simulink model "Stabilizer_QDrone"  (Simulink 9.3)
settings: Solver=ode2  StartTime=0.0  StopTime=inf  FixedStep=0.001  RelTol=1e-3  EnableMultiTasking=on
model workspace (MAT data in the model file):
  Sig = Simulink.Signal
  Sig.DataType = 'auto'
  Sig.Dimensions = -1
  Sig.DimensionsMode = 'auto'
  Sig.Complexity = 'auto'
  Sig.SampleTime = -1
  Sig.SamplingMode = 'auto'
  video_step_size = 0.06
undefined symbols (not defined in the file): datetime, HIL, m, qc_get_step_size, QDrone_, saved_data, Stabilizer_
libraries: quarc_library x28, simulink_extras x5, simulink x4
settings Model: Creator=Admin  LastModifiedBy=user  SimulationMode=external
settings SolverCC: PositivePriorityOrder=on
settings DataIOCC: SaveFormat=Dataset  SignalLoggingSaveFormat=Dataset
settings OptimizationCC: LifeSpan=auto
settings DebuggingCC: UnderspecifiedInitializationDetection=Simplified  MergeDetectMultiDrivingBlocksExec=error  ParameterPrecisionLossMsg=none  FcnCallInpInsideContextMsg=error
settings HardwareCC: ProdBitPerLong=64  ProdBitPerPointer=64  ProdBitPerSizeT=64  ProdBitPerPtrDiffT=64  ProdLargestAtomicFloat=Float  ProdIntDivRoundTo=Zero  ProdEndianess=LittleEndian  ProdWordSize=64  ProdHWDeviceType=Intel->x86-64 (Linux 64)
settings ModelReferenceCC: PropagateSignalLabelsOutOfModel=on
settings RTWCC: SystemTargetFile=quarc_linux_x64.tlc  TemplateMakefile=quarc_default_tmf  Description=QUARC Linux x64 Target (QDrone) Using Toolchain  Toolchain=QUARC linux_x64 | gmake (64-bit Windows)  BuildConfiguration=Faster Runs
settings STFCustomTargetCC: TargetPreCompLibLocation=C:\PROGRA~3\QUARC\lib\2019a\LINUX_~1\release  ConcurrentExecutionCompliant=on  SystemTargetFile=quarc_linux_x64.tlc
settings GRTTargetCC: TargetPreCompLibLocation=C:\PROGRA~3\QUARC\lib\2019a\LINUX_~1\release  ParMdlRefBuildCompliant=off  CompOptLevelCompliant=off  MatFileLogging=off  CPPClassGenCompliant=off  UseToolchainInfoCompliant=off  ExtMode=on  ExtModeMexFile=quarc_comm  ExtModeMexArgs='-w -d /tmp -uri %u -URI_Host tcpip://192.168.2.5:18001', 'tcpip://192.168.2.30:17001?retries=10', 'tcpip://192.168.2.30:17000'
settings ConfigComp: CovHtmlReporting=off

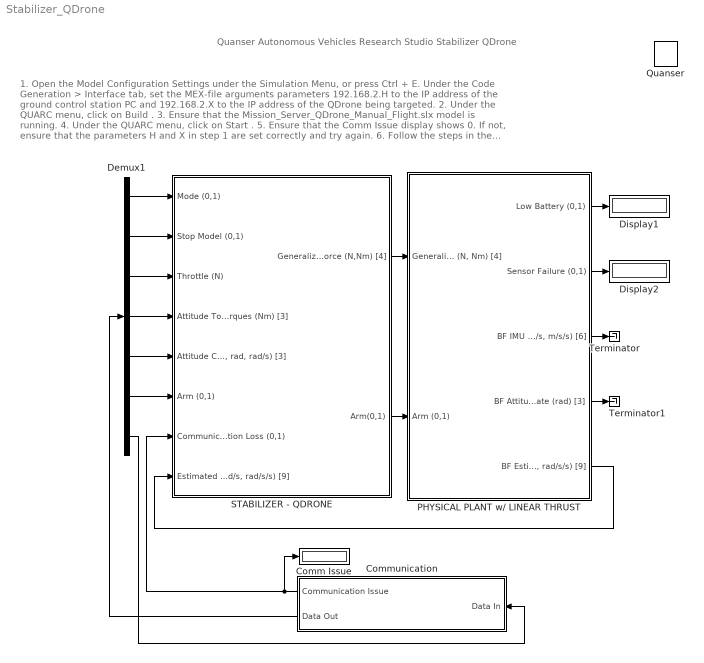
== system Stabilizer_QDrone ==
  note: Quanser Autonomous Vehicles Research Studio
      | Stabilizer QDrone
  note: 1. Open the Model Configuration Settings under the Simulation Menu, or press Ctrl + E. Under the Code Generation > Interface tab, set the MEX-file arguments parameters 192.168.2.H to the IP address of the ground control station PC and 192.168.2.X to the IP address of the QDrone being targeted.
      | 2. Under the QUARC menu, click on Build .
      | 3. Ensure that the Mission_Server_QDrone_Manual_Flight.slx model is running.
      | 4. Under the QUARC menu, click on Start .
      | 5. Ensure that the Comm Issue display shows 0. If not, ensure that the parameters H and X in step 1 are set correctly and try again.
      | 6. Follow the steps in the model to fly the drone.
      | 7. When flying is complete, stop this model first, and then the stop the Mission_Server_QDrone_Manual_Flight.slx model.
  Comm Issue : Display
  Communication : Subsystem
  Demux1 : Demux  Outputs=[1 1 1 3 3 1 1]
  Display1 : Display
      settings: Decimation=100
  Display2 : Display
      settings: Decimation=100
  PHYSICAL PLANT w/ LINEAR THRUST : Subsystem
  Quanser : quarc_library/Logos/Quanser
  STABILIZER - QDRONE : Subsystem
  Terminator : Terminator
  Terminator1 : Terminator
  wires:
  Demux1/7 -> Communication/1(Data In)
  Communication/2(Data Out) -> Demux1/1
  STABILIZER - QDRONE/1(Generalized  Force (N,Nm) [4]) -> PHYSICAL PLANT w/ LINEAR THRUST/1("Generalized Force (N, Nm) [4]")
  STABILIZER - QDRONE/2(Arm(0,1)) -> PHYSICAL PLANT w/ LINEAR THRUST/2(Arm (0,1))
  Communication/1(Communication Issue) -> Comm Issue/1, STABILIZER - QDRONE/7(Communication Loss (0,1))
  Demux1/1 -> STABILIZER - QDRONE/1(Mode (0,1))
  Demux1/2 -> STABILIZER - QDRONE/2(Stop Model (0,1))
  Demux1/3 -> STABILIZER - QDRONE/3(Throttle (N))
  Demux1/4 -> STABILIZER - QDRONE/4(Attitude Torques (Nm) [3])
  Demux1/5 -> STABILIZER - QDRONE/5("Attitude Commands (rad, rad, rad/s) [3]")
  PHYSICAL PLANT w/ LINEAR THRUST/5("BF Estimated Attitude (rad, rad/s, rad/s/s) [9]") -> STABILIZER - QDRONE/8("Estimated Attitude (rad, rad/s, rad/s/s) [9]")
  Demux1/6 -> STABILIZER - QDRONE/6(Arm (0,1))
  PHYSICAL PLANT w/ LINEAR THRUST/1(Low Battery (0,1)) -> Display1/1
  PHYSICAL PLANT w/ LINEAR THRUST/2(Sensor Failure (0,1)) -> Display2/1
  PHYSICAL PLANT w/ LINEAR THRUST/3("BF IMU Data (rad/s, m/s/s) [6]") -> Terminator/1
  PHYSICAL PLANT w/ LINEAR THRUST/4(" BF Attitude Estimate (rad) [3]") -> Terminator1/1

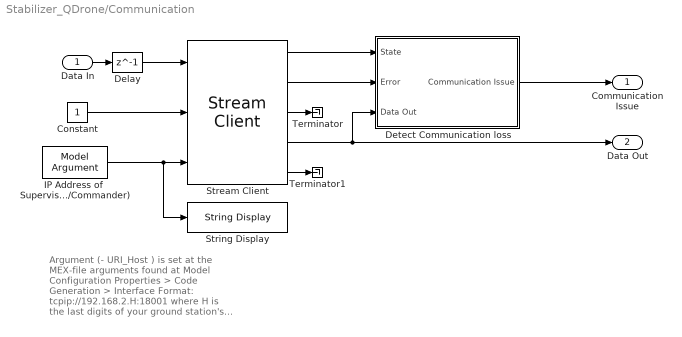
== system Stabilizer_QDrone/Communication ==
  note: Argument (- URI_Host ) is set at the MEX-file arguments found at Model Configuration Properties > Code Generation > Interface
      |
      | Format:
      | tcpip://192.168.2.H:18001
      | where H is the last digits of your ground station's IP address (use ipconfig in a command prompt to find it out).
  Data In : Inport
  Constant : Constant
  Delay : Delay  DelayLength=1
  Detect Communication loss : Subsystem
  IP Address of  Supervisory Model (Mission Operator/Commander) : quarc_library/Sources/Signals/Model Argument  argument_name=URI_Host  has_value=on  data_type_mode=Specify via dialog  data_type=char  max_length=80  variable_size=off
      settings: AttributesFormatString=(-%<argument_name>)  SourceProductName=QUARC Targets
  Stream Client : quarc_library/Communications/Basic/Stream Client  uri_source=External input port  uri=tcpip://localhost:18999  apply_uri_to_all_configs=on  send_buffer_size=1460  receive_buffer_size=1460  byte_order=little endian (Intel - LSB first)  optimization=Minimum latency  send_options=Send most recent data  receive_options=Receive most recent data  default_value=zeros(1,11)  sample_time=qc_get_step_size  active=off  implementation=Use blocking I/O in a separate thread  send_fifo_size=1  receive_fifo_size=1  send_priority=0  receive_priority=0  send_dimensions=off  receive_dimensions=off  max_dimensions=-1  data_type=Inherited via back propagation  type_expr=BusObject
      settings: SourceProductName=The database C:\Users\user\AppData\Roaming\MathWorks\MATLAB\R2017a\slblocks_master.db is locked, or a table in the database is locked. (database is locked)
  String Display : quarc_library/Strings/String Display  alignment=center  display_mode=Single line  sample_time=-1  use_new=off
      settings: SourceProductName=QUARC Targets
  Terminator : Terminator
  Terminator1 : Terminator
  Communication Issue : Outport
  Data Out : Outport  Port=2
  wires:
  Stream Client/5 -> Terminator1/1
  Constant/1 -> Stream Client/2
  Stream Client/3 -> Terminator/1
  IP Address of  Supervisory Model (Mission Operator/Commander)/1 -> String Display/1, Stream Client/3
  Stream Client/1 -> Detect Communication loss/1(State)
  Stream Client/2 -> Detect Communication loss/2(Error)
  Stream Client/4 -> Detect Communication loss/3(Data Out), Data Out/1
  Data In/1 -> Delay/1
  Delay/1 -> Stream Client/1
  Detect Communication loss/1(Communication Issue) -> Communication Issue/1

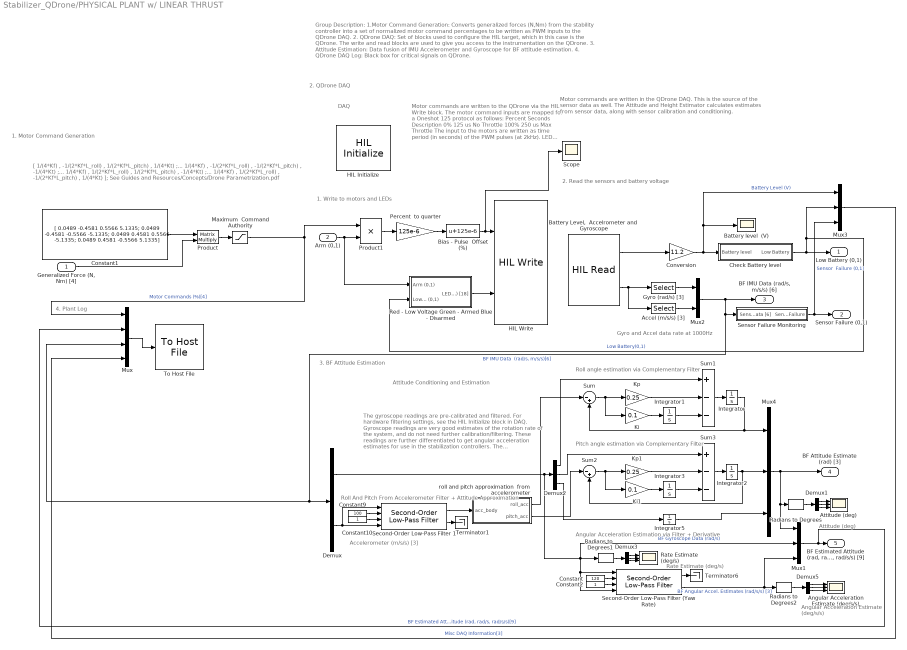
== system Stabilizer_QDrone/PHYSICAL PLANT w/ LINEAR THRUST ==
  note: Rate Estimate (deg/s)
  note: Accelerometer (m/s/s) [3]
  note: Roll And Pitch From Accelerometer Filter + Attitude Approximation
  note: Attitude Conditioning and Estimation
  note: Pitch angle estimation via Complementary Filter
  note: Roll angle estimation via Complementary Filter
  note: The gyroscope readings are pre-calibrated and filtered. For hardware filtering settings, see the HIL Initialize block in DAQ. Gyroscope readings are very good estimates of the rotation rate of the system, and do not need further calibration/filtering. These readings are further differentiated to get angular acceleration estimates for use in the stabilization controllers.
      |
      | The accelerometer readings in body reference frame are used to calculate a roll and pitch approximation. This is based on the knowledge that the gravity vector points straight down.
  note: Angular Acceleration Estimation via Filter + Derivative
  note: DAQ
  note: Motor commands are written to the QDrone via the HIL Write block. The motor command inputs are mapped for a Oneshot 125 protocol as follows:
      |
      | Percent Seconds Description
      | 0% 125 us No Throttle
      | 100% 250 us Max Throttle
      |
      | The input to the motors are written as time period (in seconds) of the PWM pulses (at 2kHz).
      |
      | LED colors can be set using a simple 3x1 ON (1) and OFF (0) vector (RGB mode).
  note: 1. Write to motors and LEDs
  note: 2. Read the sensors and battery voltage
  note: Gyro and Accel data rate at 1000Hz
  note: 1. Motor Command Generation
  note: Motor commands are written in the QDrone DAQ. This is the source of the sensor data as well. The Attitude and Height Estimator calculates estimates from sensor data, along with sensor calibration and conditioning.
  note: Angular Acceleration
      | Estimate (deg/s/s)
  note: Attitude (deg)
  note: [ 1/(4*Kf) , -1/(2*Kf*L_roll) , 1/(2*Kf*L_pitch) , 1/(4*Kt) ;...
      | 1/(4*Kf) , -1/(2*Kf*L_roll) , -1/(2*Kf*L_pitch) , -1/(4*Kt) ;...
      | 1/(4*Kf) , 1/(2*Kf*L_roll) , 1/(2*Kf*L_pitch) , -1/(4*Kt) ;...
      | 1/(4*Kf) , 1/(2*Kf*L_roll) , -1/(2*Kf*L_pitch) , 1/(4*Kt) ];
      |
      | See Guides and Resources/Concepts/Drone Parametrization.pdf
  note: 4. Plant Log
  note: Group Description:
      |
      | 1.Motor Command Generation: Converts generalized forces (N,Nm) from the stability controller into a set of normalized motor command percentages to be written as PWM inputs to the QDrone DAQ.
      | 2. QDrone DAQ: Set of blocks used to configure the HIL target, which in this case is the QDrone. The write and read blocks are used to give you access to the instrumentation on the QDrone.
      | 3. Attitude Estimation: Data fusion of IMU Accelerometer and Gyroscope for BF attitude estimation.
      | 4. QDrone DAQ Log: Black box for critical signals on QDrone.
  note: 2. QDrone DAQ
  note: 3. BF Attitude Estimation
  "Generalized Force (N, Nm) [4]" : Inport
  Arm (0,1) : Inport  Port=2
  Accel (m/s/s) [3] : Selector  InputPortWidth=6  IndexOptions=Index vector (dialog)  Indices=[4:6]  OutputSizes=1
  Angular Acceleration Estimate (deg/s/s) : Scope  NumInputPorts=3
  Attitude (deg) : Scope  NumInputPorts=3
  "Battery Level,  Accelrometer and  Gyroscope" : quarc_library/Data Acquisition/Generic/Immediate I//O/HIL Read  Priority=1  object_name=HIL-1  analog_channels=[4]  encoder_channels=[]  digital_channels=[]  other_channels=[3000:3002 4000:4002]  sample_time=qc_get_step_size  active=on  vector_output=on  data_type_mode=Inherit via back propagation  encoder_data_type=double  digital_data_type=boolean
      settings: SourceProductName=The database C:\Users\user\AppData\Roaming\MathWorks\MATLAB\R2017a\slblocks_master.db is locked, or a table in the database is locked. (database is locked)
  Battery level  (V) : Scope
  Bias - Pulse  Offset (%) : Bias  Bias=125e-6
  Check Battery level : Subsystem
  Constant : Constant  Value=120
  Constant1 : Constant  Value=|
      | [ 0.0489   -0.4581    0.5566    5.1335;
      |   0.0489   -0.4581   -0.5566   -5.1335;
      |   0.0489    0.4581    0.5566   -5.1335;
      |   0.0489    0.4581   -0.5566    5.1335]
  Constant10 : Constant
  Constant2 : Constant
  Constant9 : Constant  Value=100
  Conversion : Gain  Gain=11.2
  Demux : Demux  Outputs=[3 3]
  Demux{1..3,5} (4 alike) : Demux  Outputs=3
  Gyro (rad/s) [3] : Selector  InputPortWidth=6  IndexOptions=Index vector (dialog)  Indices=[1:3]  OutputSizes=1
  HIL Initialize : quarc_library/Data Acquisition/Generic/Configuration/HIL Initialize  object_name=HIL-1  board_type=qdrone  board_number=0  board_options=gyro_fs=2000;gyro_rate=1000;gyro_os=4;accel_fs=16;accel_rate=400;accel_os=4;baro_os=4096  exclusive=off  active=on  hardware_clocks=[]  clock_modes=[]  initial_clock_frequencies=[]  set_clock_params_at_start=off  set_clock_params_at_switch_in=off  set_clock_frequencies_at_start=off  set_clock_frequencies_at_switch_in=off  analog_input_channels=[0:4]  analog_input_configurations=[]  analog_input_maximums=[3.3]  analog_input_minimums=[0]  set_analog_input_params_at_start=off  set_analog_input_params_at_switch_in=off  analog_output_channels=[]  analog_output_maximums=[]  analog_output_minimums=[]  initial_analog_outputs=[]  final_analog_outputs=[]  watchdog_analog_outputs=[]  set_analog_output_params_at_start=off  set_analog_output_params_at_switch_in=off  set_analog_outputs_at_start=off  set_analog_outputs_at_switch_in=off  set_analog_outputs_at_terminate=off  set_analog_outputs_at_switch_out=off  set_analog_outputs_on_watchdog=off  digital_input_channels=[]  digital_output_channels=[5:7 9:23]  digital_output_configuration=[]  initial_digital_outputs=[0]  final_digital_outputs=[0]  watchdog_digital_outputs=[]  set_digital_output_params_at_start=off  set_digital_output_params_at_switch_in=off  set_digital_outputs_at_start=on  set_digital_outputs_at_switch_in=off  set_digital_outputs_at_terminate=on  set_digital_outputs_at_switch_out=off  set_digital_outputs_on_watchdog=off  encoder_channels=[0:2]  quadrature=[4]  encoder_filter_frequency=50e6/1  initial_encoder_counts=[0]  set_encoder_params_at_start=on  set_encoder_params_at_switch_in=off  set_encoder_counts_at_start=on  set_encoder_counts_at_switch_in=off  pwm_channels=[0:3]  pwm_modes=[4]  pwm_frequency=2000  pwm_configuration=[0]  pwm_alignment=[0]  pwm_polarity=[1]  pwm_leading_deadband=[]  pwm_trailing_deadband=[]  initial_pwm_outputs=[0]  final_pwm_outputs=[0]  watchdog_pwm_outputs=[0]  set_pwm_params_at_start=on  set_pwm_params_at_switch_in=off  set_pwm_outputs_at_start=on  set_pwm_outputs_at_switch_in=off  set_pwm_outputs_at_terminate=on  set_pwm_outputs_at_switch_out=off  set_pwm_outputs_on_watchdog=off  other_output_channels=[]  initial_other_outputs=[]  final_other_outputs=[]  watchdog_other_outputs=[]  set_other_outputs_at_start=off  set_other_outputs_at_switch_in=off  set_other_outputs_at_terminate=off  set_other_outputs_at_switch_out=off  set_other_outputs_on_watchdog=off
      settings: SourceProductName=The database C:\Users\user\AppData\Roaming\MathWorks\MATLAB\R2017a\slblocks_master.db is locked, or a table in the database is locked. (database is locked)
  HIL Write : quarc_library/Data Acquisition/Generic/Immediate I//O/HIL Write  object_name=HIL-1  analog_channels=[]  pwm_channels=[0:3]  digital_channels=[5:7 9:23]  other_channels=[]  sample_time=-1  active=off  vector_input=on
      settings: SourceProductName=The database C:\Users\user\AppData\Roaming\MathWorks\MATLAB\R2017a\slblocks_master.db is locked, or a table in the database is locked. (database is locked)
  Integrator{,1..3,5} (5 alike) : Integrator
  Ki : Gain  Gain=0.1
  Ki1 : Gain  Gain=0.1
  Kp : Gain  Gain=0.25
  Kp1 : Gain  Gain=0.25
  "Maximum  Command Authority " : Saturate  UpperLimit=[1 1 1 1]  LowerLimit=[0 0 0 0]
  Mux : Mux
  Mux1 : Mux  Inputs=3
  Mux2 : Mux  Inputs=2
  Mux3 : Mux  Inputs=3
  Mux4 : Mux  Inputs=3
  Percent  to quarter : Gain  Gain=125e-6
  Product : Product  Multiplication=Matrix(*)
  Product1 : Product
  Radians to Degrees : simulink_extras/Transformations/Radians to Degrees
  Radians to Degrees1 : simulink_extras/Transformations/Radians to Degrees
  Radians to Degrees2 : simulink_extras/Transformations/Radians to Degrees
  Rate Estimate (deg/s) : Scope  NumInputPorts=3
  Red - Low Voltage Green - Armed Blue - Disarmed : Subsystem
  Scope : Scope
  Second-Order Low-Pass Filter (Yaw Rate) : quarc_library/Continuous/Second-Order Low-Pass Filter  params_source=External (input ports)  input_width=200  input_zeta=1  input_init=0
      settings: SourceProductName=The database C:\Users\user\AppData\Roaming\MathWorks\MATLAB\R2017a\slblocks_master.db is locked, or a table in the database is locked. (database is locked)
  Second-Order Low-Pass Filter 1 : quarc_library/Continuous/Second-Order Low-Pass Filter  params_source=External (input ports)  input_width=50  input_zeta=1  input_init=0
      settings: SourceProductName=The database C:\Users\user\AppData\Roaming\MathWorks\MATLAB\R2017a\slblocks_master.db is locked, or a table in the database is locked. (database is locked)
  Sensor Failure Monitoring : Subsystem
  Sum : Sum  Inputs=|-+
  Sum1 : Sum  Inputs=+--
  Sum2 : Sum  Inputs=|-+
  Sum3 : Sum  Inputs=+--
  Terminator1 : Terminator
  Terminator6 : Terminator
  To Host File : quarc_library/Sinks/To Host/To Host File  file_name=saved_data/%m/QDrone_%{char(datetime)}.mat  variable_name=QDrone_data  decimation=1  sample_time=-1  file_format=MAT-file v.5  options=No header or footer  append=off  final_file_name=saved_data/Stabilizer_QDrone/QDrone_05-Nov-2026 13-08-41.mat  bitrate=2000000
      settings: SourceProductName=The database C:\Users\user\AppData\Roaming\MathWorks\MATLAB\R2017a\slblocks_master.db is locked, or a table in the database is locked. (database is locked)
  roll and pitch approximation  from accelerometer : MATLAB Function  TreatAsAtomicUnit=on
  Low Battery (0,1) : Outport
  Sensor Failure (0,1) : Outport  Port=2
  "BF IMU Data (rad/s, m/s/s) [6]" : Outport  Port=3
  " BF Attitude Estimate (rad) [3]" : Outport  Port=4
  "BF Estimated Attitude (rad, rad/s, rad/s/s) [9]" : Outport  Port=5
  wires:
  Mux3/1 -> Mux/4  "Misc DAQ Information[3]"
  Check Battery level/1(Low Battery) -> Low Battery (0,1)/1, Red - Low Voltage Green - Armed Blue - Disarmed/2(Low Battery (0,1)), Mux3/2  "Low Battery(0,1)"
  Arm (0,1)/1 -> Product1/2, Red - Low Voltage Green - Armed Blue - Disarmed/1(Arm (0,1))
  Mux1/1 -> "BF Estimated Attitude (rad, rad/s, rad/s/s) [9]"/1, Mux/2  "BF Estimated Attitude (rad, rad/s, rad/s/s)[9]"
  Demux3/1 -> Rate Estimate (deg/s)/1
  Demux3/2 -> Rate Estimate (deg/s)/2
  Radians to Degrees1/1 -> Demux3/1
  Demux/1 -> Demux2/1, Second-Order Low-Pass Filter (Yaw Rate)/1, Second-Order Low-Pass Filter (Yaw Rate)/4, Radians to Degrees1/1, Mux1/2  "BF Gyroscope Data (rad/s)"
  Demux3/3 -> Rate Estimate (deg/s)/3
  Second-Order Low-Pass Filter (Yaw Rate)/2 -> Mux1/3, Radians to Degrees2/1  "BF Angular Accel. Estimates (rad/s/s) [3]"
  Second-Order Low-Pass Filter 1/2 -> Terminator1/1
  roll and pitch approximation  from accelerometer/2(pitch_acc) -> Sum2/1
  Kp/1 -> Sum1/2
  Constant10/1 -> Second-Order Low-Pass Filter 1/3
  Demux/2 -> Second-Order Low-Pass Filter 1/4, Second-Order Low-Pass Filter 1/1
  Constant2/1 -> Second-Order Low-Pass Filter (Yaw Rate)/3
  Sum/1 -> Kp/1, Ki/1
  Demux2/3 -> Integrator5/1
  roll and pitch approximation  from accelerometer/1(roll_acc) -> Sum/1
  Second-Order Low-Pass Filter 1/1 -> roll and pitch approximation  from accelerometer/1(acc_body)
  Second-Order Low-Pass Filter (Yaw Rate)/1 -> Terminator6/1
  Constant9/1 -> Second-Order Low-Pass Filter 1/2
  Mux4/1 -> " BF Attitude Estimate (rad) [3]"/1, Mux1/1, Radians to Degrees/1
  Ki1/1 -> Integrator3/1
  Integrator1/1 -> Sum1/3
  Sum1/1 -> Integrator/1
  Sum3/1 -> Integrator2/1
  Sum2/1 -> Ki1/1, Kp1/1
  Kp1/1 -> Sum3/2
  Integrator/1 -> Mux4/1, Sum/2
  Constant/1 -> Second-Order Low-Pass Filter (Yaw Rate)/2
  Demux2/1 -> Sum1/1
  Ki/1 -> Integrator1/1
  Integrator5/1 -> Mux4/3
  Integrator2/1 -> Mux4/2, Sum2/2
  Integrator3/1 -> Sum3/3
  Demux2/2 -> Sum3/1
  Mux2/1 -> "BF IMU Data (rad/s, m/s/s) [6]"/1, Sensor Failure Monitoring/1(Sensor Data [6]), Demux/1, Mux/3  "BF IMU Data  (rad/s, m/s/s)[6]"
  Sensor Failure Monitoring/1(Sensor Failure) -> Mux3/3, Sensor Failure (0,1)/1  "Sensor  Failure (0,1)"
  Gyro (rad/s) [3]/1 -> Mux2/1
  "Battery Level,  Accelrometer and  Gyroscope"/1 -> Conversion/1
  "Battery Level,  Accelrometer and  Gyroscope"/2 -> Gyro (rad/s) [3]/1, Accel (m/s/s) [3]/1
  Percent  to quarter/1 -> Bias - Pulse  Offset (%)/1
  Bias - Pulse  Offset (%)/1 -> Scope/1, HIL Write/1
  Red - Low Voltage Green - Armed Blue - Disarmed/1(LEDs (%) [18]) -> HIL Write/2
  Product1/1 -> Percent  to quarter/1
  Accel (m/s/s) [3]/1 -> Mux2/2
  Mux/1 -> To Host File/1
  Product/1 -> "Maximum  Command Authority "/1
  "Generalized Force (N, Nm) [4]"/1 -> Product/2
  Constant1/1 -> Product/1
  Conversion/1 -> Battery level  (V)/1, Mux3/1, Check Battery level/1(Battery level)  "Battery Level (V)"
  "Maximum  Command Authority "/1 -> Product1/1, Mux/1  "Motor Commands (%)[4]"
  Radians to Degrees2/1 -> Demux5/1
  Radians to Degrees/1 -> Demux1/1
  Demux5/3 -> Angular Acceleration Estimate (deg/s/s)/3
  Demux5/2 -> Angular Acceleration Estimate (deg/s/s)/2
  Demux5/1 -> Angular Acceleration Estimate (deg/s/s)/1
  Demux1/3 -> Attitude (deg)/3
  Demux1/2 -> Attitude (deg)/2
  Demux1/1 -> Attitude (deg)/1

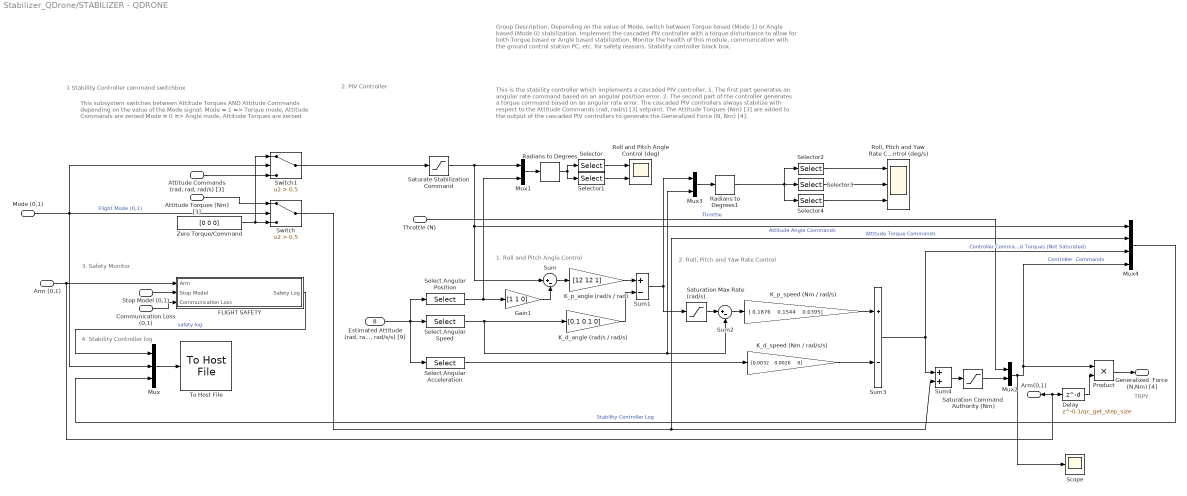
== system Stabilizer_QDrone/STABILIZER - QDRONE ==
  note: 2. PIV Controller
  note: 4. Stability Controller log
  note: 1 Stability Controller command switchbox
  note: Group Description:
      |
      | Depending on the value of Mode, switch between Torque based (Mode 1) or Angle based (Mode 0) stabilization.
      | Implement the cascaded PIV controller with a torque disturbance to allow for both Torque based or Angle based stabilization.
      | Monitor the health of this module, communication with the ground control station PC, etc. for safety reasons.
      | Stability controller black box.
  note: TRPY
  note: 2. Roll, Pitch and Yaw Rate Control
  note: 1. Roll and Pitch Angle Control
  note: This is the stability controller which implements a cascaded PIV controller.
      | 1. The first part generates an angular rate command based on an angular position error.
      | 2. The second part of the controller generates a torque command based on an angular rate error.
      |
      | The cascaded PIV controllers always stabilize with respect to the Attitude Commands (rad, rad/s) [3] setpoint. The Attitude Torques (Nm) [3] are added to the output of the cascaded PIV controllers to generate the Generalized Force (N, Nm) [4].
  note: This subsystem switches between Attitude Torques AND Attitude Commands depending on
      | the value of the Mode signal:
      | Mode = 1	=> 		Torque mode, Attitude Commands are zeroed
      | Mode = 0	=> 		Angle mode, Attitude Torques are zeroed
  note: 3. Safety Monitor
  Mode (0,1) : Inport
  Stop Model (0,1) : Inport  Port=2
  Throttle (N) : Inport  Port=3
  Attitude Torques (Nm) [3] : Inport  Port=4
  "Attitude Commands (rad, rad, rad/s) [3]" : Inport  Port=5
  Arm (0,1) : Inport  Port=6
  Communication Loss (0,1) : Inport  Port=7
  "Estimated Attitude (rad, rad/s, rad/s/s) [9]" : Inport  Port=8
  Delay : Delay  DelayLength=0.1/qc_get_step_size
  FLIGHT SAFETY : Subsystem
  Gain1 : Gain  Gain=[1 1 0]
  K_d_angle (rad/s / rad/s) : Gain  Gain=[0.1 0.1 0]
  K_d_speed (Nm / rad/s/s) : Gain  Gain="[0.0032    0.0026     0]"
  K_p_angle (rad/s / rad) : Gain  Gain=[12 12 1]
  K_p_speed (Nm / rad/s) : Gain  Gain="[ 0.1876    0.1544    0.0395]"
  Mux : Mux  Inputs=3
  Mux1 : Mux  Inputs=2
  Mux2 : Mux  Inputs=2
  Mux3 : Mux  Inputs=2
  Mux4 : Mux
  Product : Product
  Radians to Degrees : simulink_extras/Transformations/Radians to Degrees
  Radians to Degrees1 : simulink_extras/Transformations/Radians to Degrees
  Roll and Pitch Angle Control (deg) : Scope  NumInputPorts=2
  "Roll, Pitch and Yaw Rate Control (deg/s)" : Scope  NumInputPorts=3
  Saturate Stabilization Command : Saturate  UpperLimit=[pi/4 pi/4 10*pi/18]  LowerLimit=[-pi/4 -pi/4 -10*pi/18]
  Saturation Command  Authority (Nm) : Saturate  UpperLimit=[1.0915 0.8984 0.0984]  LowerLimit=-[1.0915 0.8984 0.0984]
  Saturation Max Rate  (rad/s) : Saturate  UpperLimit=10*pi/3*[1 1 1]  LowerLimit=-10*pi/3*[1 1 1]
  Scope : Scope
  Select Angular Acceleration : Selector  InputPortWidth=9  IndexOptions=Index vector (dialog)  Indices=[7:9]  OutputSizes=1
  Select Angular Speed : Selector  InputPortWidth=9  IndexOptions=Index vector (dialog)  Indices=[4:6]  OutputSizes=1
  Select Angular Position : Selector  InputPortWidth=9  IndexOptions=Index vector (dialog)  Indices=[1:3]  OutputSizes=1
  Selector : Selector  InputPortWidth=6  IndexOptions=Index vector (dialog)  Indices=[1 4]  OutputSizes=1
  Selector1 : Selector  InputPortWidth=6  IndexOptions=Index vector (dialog)  Indices=[2 5]  OutputSizes=1
  Selector2 : Selector  InputPortWidth=6  IndexOptions=Index vector (dialog)  Indices=[1 4]  OutputSizes=1
  Selector3 : Selector  InputPortWidth=6  IndexOptions=Index vector (dialog)  Indices=[2 5]  OutputSizes=1
  Selector4 : Selector  InputPortWidth=6  IndexOptions=Index vector (dialog)  Indices=[3 6]  OutputSizes=1
  Sum : Sum  Inputs=|+-
  Sum1 : Sum  Inputs=+-
  Sum2 : Sum  Inputs=|+-
  Sum3 : Sum  Inputs=+-
  Sum4 : Sum
  Switch : Switch  Criteria=u2 > Threshold  Threshold=0.5
  Switch1 : Switch  Criteria=u2 > Threshold  Threshold=0.5
  To Host File : quarc_library/Sinks/To Host/To Host File  file_name=saved_data/%m/Stabilizer_%{char(datetime)}.mat  variable_name=stabilizer_data  decimation=1  sample_time=-1  file_format=MAT-file v.5  options=No header or footer  append=off  final_file_name=saved_data/Stabilizer_QDrone/Stabilizer_05-Nov-2026 13-08-41.mat  bitrate=2000000
      settings: SourceProductName=The database C:\Users\user\AppData\Roaming\MathWorks\MATLAB\R2017a\slblocks_master.db is locked, or a table in the database is locked. (database is locked)
  Zero Torque/Command : Constant  Value=[0 0 0]
  Generalized  Force (N,Nm) [4] : Outport
  Arm(0,1) : Outport  Port=2
  wires:
  Product/1 -> Generalized  Force (N,Nm) [4]/1
  Stop Model (0,1)/1 -> FLIGHT SAFETY/2(Stop Model)
  Communication Loss (0,1)/1 -> FLIGHT SAFETY/3(Communication Loss)
  Mux/1 -> To Host File/1
  Mux4/1 -> Mux/3  "Stability Controller Log"
  Mode (0,1)/1 -> Switch/2, Switch1/2, Mux/2  "Flight Mode (0,1)"
  FLIGHT SAFETY/1(Safety Log) -> Mux/1  "safety log"
  K_p_speed (Nm / rad/s)/1 -> Sum3/1
  Sum/1 -> K_p_angle (rad/s / rad)/1
  K_d_speed (Nm / rad/s/s)/1 -> Sum3/2
  Arm (0,1)/1 -> Arm(0,1)/1, Delay/1, FLIGHT SAFETY/1(Arm)
  Mux3/1 -> Radians to Degrees1/1
  Sum1/1 -> Saturation Max Rate  (rad/s)/1, Mux3/1
  Saturate Stabilization Command/1 -> Mux1/1, Sum/1, Mux4/1  "Attitude Angle Commands"
  Mux2/1 -> Scope/1, Mux4/4, Product/1  "Controller  Commands"
  Select Angular Position/1 -> Mux1/2, Gain1/1
  Sum2/1 -> K_p_speed (Nm / rad/s)/1
  Throttle (N)/1 -> Mux2/1  "Throttle"
  Selector1/1 -> Roll and Pitch Angle Control (deg)/2
  Switch/1 -> Mux4/2, Sum4/2  "Attitude Torque Commands"
  Radians to Degrees1/1 -> Selector2/1, Selector4/1, Selector3/1
  "Estimated Attitude (rad, rad/s, rad/s/s) [9]"/1 -> Select Angular Position/1, Select Angular Acceleration/1, Select Angular Speed/1
  Mux1/1 -> Radians to Degrees/1
  Selector3/1 -> "Roll, Pitch and Yaw Rate Control (deg/s)"/2
  Sum4/1 -> Saturation Command  Authority (Nm)/1
  Sum3/1 -> Mux4/3, Sum4/1  "Controller Command Torques (Not Saturated)"
  Saturation Command  Authority (Nm)/1 -> Mux2/2
  Gain1/1 -> Sum/2
  Select Angular Acceleration/1 -> K_d_speed (Nm / rad/s/s)/1
  Switch1/1 -> Saturate Stabilization Command/1
  Saturation Max Rate  (rad/s)/1 -> Sum2/1
  Selector4/1 -> "Roll, Pitch and Yaw Rate Control (deg/s)"/3
  K_p_angle (rad/s / rad)/1 -> Sum1/1
  Select Angular Speed/1 -> Sum2/2, Mux3/2, K_d_angle (rad/s / rad/s)/1
  Selector/1 -> Roll and Pitch Angle Control (deg)/1
  Selector2/1 -> "Roll, Pitch and Yaw Rate Control (deg/s)"/1
  K_d_angle (rad/s / rad/s)/1 -> Sum1/2
  Radians to Degrees/1 -> Selector/1, Selector1/1
  "Attitude Commands (rad, rad, rad/s) [3]"/1 -> Switch1/3
  Attitude Torques (Nm) [3]/1 -> Switch/1
  Zero Torque/Command/1 -> Switch1/1, Switch/3
  Delay/1 -> Product/2

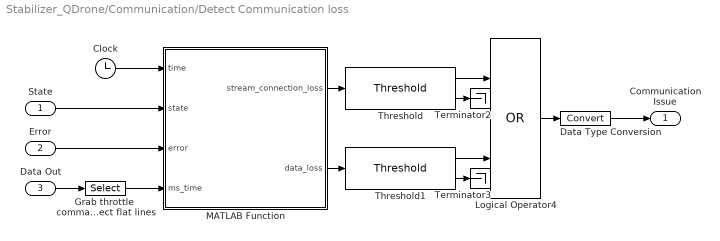
== system Stabilizer_QDrone/Communication/Detect Communication loss ==
  State : Inport
  Error : Inport  Port=2
  Data Out : Inport  Port=3
  Clock : Clock
  Data Type Conversion : DataTypeConversion
  Grab throttle  command to  detect flat lines : Selector  InputPortWidth=11  IndexOptions=Index vector (dialog)  Indices=[11]  OutputSizes=1
  Logical Operator4 : Logic  Operator=OR  AllPortsSameDT=off  OutDataTypeStr=boolean
  MATLAB Function : MATLAB Function  TreatAsAtomicUnit=on
  Terminator2 : Terminator
  Terminator3 : Terminator
  Threshold : quarc_library/Discontinuities/Threshold  operator=>=  param_src=Specify via dialog  threshold=0.5  duration=0.1
      settings: SourceProductName=QUARC Targets
  Threshold1 : quarc_library/Discontinuities/Threshold  operator=>=  param_src=Specify via dialog  threshold=0.5  duration=0.5
      settings: SourceProductName=QUARC Targets
  Communication Issue : Outport
  wires:
  Threshold/1 -> Logical Operator4/1
  Error/1 -> MATLAB Function/3(error)
  MATLAB Function/1(stream_connection_loss) -> Threshold/1
  State/1 -> MATLAB Function/2(state)
  Clock/1 -> MATLAB Function/1(time)
  Logical Operator4/1 -> Data Type Conversion/1
  Threshold1/2 -> Terminator3/1
  Threshold/2 -> Terminator2/1
  Data Type Conversion/1 -> Communication Issue/1
  MATLAB Function/2(data_loss) -> Threshold1/1
  Data Out/1 -> Grab throttle  command to  detect flat lines/1
  Threshold1/1 -> Logical Operator4/2
  Grab throttle  command to  detect flat lines/1 -> MATLAB Function/4(ms_time)

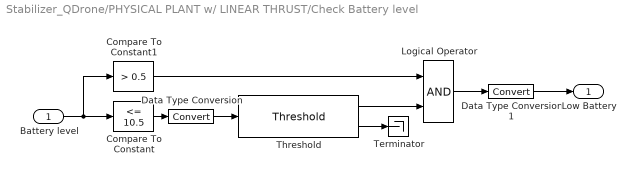
== system Stabilizer_QDrone/PHYSICAL PLANT w/ LINEAR THRUST/Check Battery level ==
  Battery level : Inport
  Compare To Constant : simulink/Logic and Bit Operations/Compare To Constant  relop=<=  const=10.5  OutDataTypeStr=boolean
  Compare To Constant1 : simulink/Logic and Bit Operations/Compare To Constant  relop=>  const=0.5  OutDataTypeStr=boolean
  Data Type Conversion : DataTypeConversion
  Data Type Conversion1 : DataTypeConversion
  Logical Operator : Logic  AllPortsSameDT=off  OutDataTypeStr=boolean
  Terminator : Terminator
  Threshold : quarc_library/Discontinuities/Threshold  operator=>=  param_src=Specify via dialog  threshold=0.5  duration=0.1
      settings: SourceProductName=The database C:\Users\user\AppData\Roaming\MathWorks\MATLAB\R2017a\slblocks_master.db is locked, or a table in the database is locked. (database is locked)
  Low Battery : Outport
  wires:
  Data Type Conversion1/1 -> Low Battery/1
  Data Type Conversion/1 -> Threshold/1
  Compare To Constant/1 -> Data Type Conversion/1
  Compare To Constant1/1 -> Logical Operator/1
  Logical Operator/1 -> Data Type Conversion1/1
  Threshold/1 -> Logical Operator/2
  Battery level/1 -> Compare To Constant/1, Compare To Constant1/1
  Threshold/2 -> Terminator/1

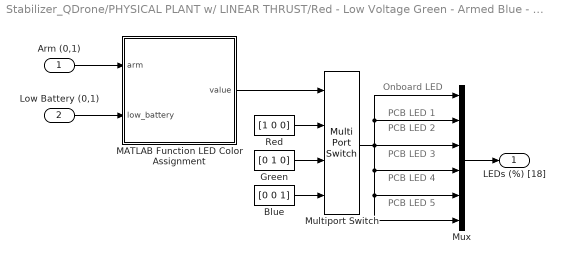
== system Stabilizer_QDrone/PHYSICAL PLANT w/ LINEAR THRUST/Red - Low Voltage Green - Armed Blue - Disarmed ==
  note: Onboard LED
  note: PCB LED 4
  note: PCB LED 5
  note: PCB LED 1
  note: PCB LED 2
  note: PCB LED 3
  Arm (0,1) : Inport
  Low Battery (0,1) : Inport  Port=2
  Blue : Constant  Value=[0 0 1]
  Green : Constant  Value=[0 1 0]
  MATLAB Function LED Color Assignment : MATLAB Function  TreatAsAtomicUnit=on
  Multiport Switch : MultiPortSwitch
  Mux : Mux  Inputs=[3 3 3 3 3 3]
  Red : Constant  Value=[1 0 0]
  LEDs (%) [18] : Outport
  wires:
  Mux/1 -> LEDs (%) [18]/1
  Low Battery (0,1)/1 -> MATLAB Function LED Color Assignment/2(low_battery)
  MATLAB Function LED Color Assignment/1(value) -> Multiport Switch/1
  Arm (0,1)/1 -> MATLAB Function LED Color Assignment/1(arm)
  Blue/1 -> Multiport Switch/4
  Green/1 -> Multiport Switch/3
  Red/1 -> Multiport Switch/2
  Multiport Switch/1 -> Mux/1, Mux/2, Mux/3, Mux/6, Mux/5, Mux/4

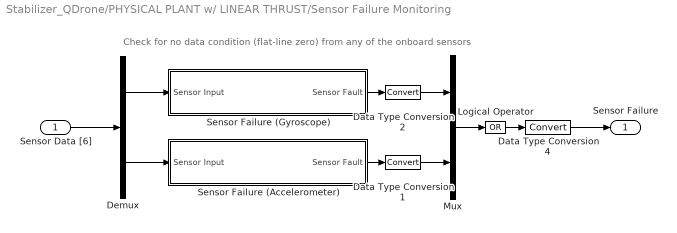
== system Stabilizer_QDrone/PHYSICAL PLANT w/ LINEAR THRUST/Sensor Failure Monitoring ==
  note: Check for no data condition (flat-line zero) from any of the onboard sensors
  Sensor Data [6] : Inport
  Data Type Conversion1 : DataTypeConversion
  Data Type Conversion2 : DataTypeConversion
  Data Type Conversion4 : DataTypeConversion
  Demux : Demux  Outputs=[3 3]
  Logical Operator : Logic  Operator=OR  Inputs=1  AllPortsSameDT=off  OutDataTypeStr=boolean
  Mux : Mux  Inputs=2
  Sensor Failure (Accelerometer) : Subsystem
  Sensor Failure (Gyroscope) : Subsystem
  Sensor Failure : Outport
  wires:
  Data Type Conversion4/1 -> Sensor Failure/1
  Logical Operator/1 -> Data Type Conversion4/1
  Demux/1 -> Sensor Failure (Gyroscope)/1(Sensor Input)
  Sensor Data [6]/1 -> Demux/1
  Data Type Conversion1/1 -> Mux/2
  Data Type Conversion2/1 -> Mux/1
  Mux/1 -> Logical Operator/1
  Sensor Failure (Accelerometer)/1(Sensor Fault) -> Data Type Conversion1/1
  Sensor Failure (Gyroscope)/1(Sensor Fault) -> Data Type Conversion2/1
  Demux/2 -> Sensor Failure (Accelerometer)/1(Sensor Input)

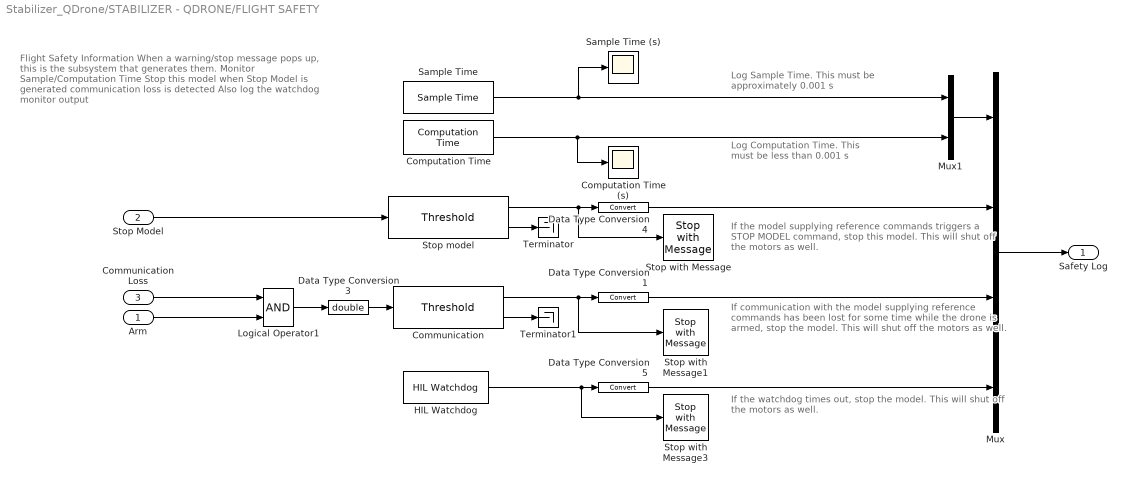
== system Stabilizer_QDrone/STABILIZER - QDRONE/FLIGHT SAFETY ==
  note: Flight Safety Information
      |
      | When a warning/stop message pops up, this is the subsystem
      | that generates them.
      |
      | Monitor Sample/Computation Time
      | Stop this model
      | when Stop Model is generated
      | communication loss is detected
      | Also log the watchdog monitor output
  note: Log Sample Time. This must be approximately 0.001 s
  note: Log Computation Time. This must be less than 0.001 s
  note: If the model supplying reference commands triggers a STOP MODEL command, stop this model. This will shut off the motors as well.
  note: If communication with the model supplying reference commands has been lost for some time while the drone is armed, stop the model. This will shut off the motors as well.
  note: If the watchdog times out, stop the model. This will shut off the motors as well.
  Arm : Inport
  Stop Model : Inport  Port=2
  Communication Loss : Inport  Port=3
  Communication : quarc_library/Discontinuities/Threshold  operator=>=  param_src=Specify via dialog  threshold=0.5  duration=1
      settings: SourceProductName=The database C:\Users\user\AppData\Roaming\MathWorks\MATLAB\R2017a\slblocks_master.db is locked, or a table in the database is locked. (database is locked)
  Computation Time : quarc_library/Sources/Time/Computation Time  sample_time=qc_get_step_size  use_model=on  use_cpu_time=off
      settings: SourceProductName=The database C:\Users\user\AppData\Roaming\MathWorks\MATLAB\R2017a\slblocks_master.db is locked, or a table in the database is locked. (database is locked)
  Computation Time (s) : Scope
  Data Type Conversion1 : DataTypeConversion
  Data Type Conversion3 : DataTypeConversion  OutDataTypeStr=double
  Data Type Conversion4 : DataTypeConversion
  Data Type Conversion5 : DataTypeConversion
  HIL Watchdog : quarc_library/Data Acquisition/Generic/Watchdog/HIL Watchdog  object_name=HIL-1  timeout=0.1  sample_time=qc_get_step_size  active=off
      settings: AttributesFormatString=(%<object_name>)  SourceProductName=QUARC Targets
  Logical Operator1 : Logic  AllPortsSameDT=off  OutDataTypeStr=boolean
  Mux : Mux
  Mux1 : Mux  Inputs=2
  Sample Time : quarc_library/Sources/Time/Sample Time  Priority=-99  sample_time=qc_get_step_size
      settings: SourceProductName=The database C:\Users\user\AppData\Roaming\MathWorks\MATLAB\R2017a\slblocks_master.db is locked, or a table in the database is locked. (database is locked)
  Sample Time (s) : Scope
  Stop model : quarc_library/Discontinuities/Threshold  operator=>=  param_src=Specify via dialog  threshold=0.5  duration=0.1
      settings: SourceProductName=The database C:\Users\user\AppData\Roaming\MathWorks\MATLAB\R2017a\slblocks_master.db is locked, or a table in the database is locked. (database is locked)
  Stop with Message : quarc_library/Sinks/Error Handling/Stop with Message  message_type=Fixed error message  message_icon=Information  message=QDrone Stabilizer: Commander Terminated
      settings: SourceProductName=The database C:\Users\user\AppData\Roaming\MathWorks\MATLAB\R2017a\slblocks_master.db is locked, or a table in the database is locked. (database is locked)
  Stop with Message1 : quarc_library/Sinks/Error Handling/Stop with Message  message_type=Fixed error message  message_icon=Warning  message=QDrone Stabilizer: Communication with Commander lost
      settings: SourceProductName=The database C:\Users\user\AppData\Roaming\MathWorks\MATLAB\R2017a\slblocks_master.db is locked, or a table in the database is locked. (database is locked)
  Stop with Message3 : quarc_library/Sinks/Error Handling/Stop with Message  message_type=Fixed error message  message_icon=Information  message=QDrone Stabilizer: HIL Watchdog timer expired
      settings: SourceProductName=The database C:\Users\user\AppData\Roaming\MathWorks\MATLAB\R2017a\slblocks_master.db is locked, or a table in the database is locked. (database is locked)
  Terminator : Terminator
  Terminator1 : Terminator
  Safety Log : Outport
  wires:
  Mux/1 -> Safety Log/1
  Computation Time/1 -> Computation Time (s)/1, Mux1/2
  Sample Time/1 -> Sample Time (s)/1, Mux1/1
  Data Type Conversion4/1 -> Mux/2
  HIL Watchdog/1 -> Stop with Message3/1, Data Type Conversion5/1
  Stop model/2 -> Terminator/1
  Stop model/1 -> Data Type Conversion4/1, Stop with Message/1
  Stop Model/1 -> Stop model/1
  Communication/2 -> Terminator1/1
  Logical Operator1/1 -> Data Type Conversion3/1
  Data Type Conversion1/1 -> Mux/3
  Arm/1 -> Logical Operator1/2
  Communication/1 -> Data Type Conversion1/1, Stop with Message1/1
  Data Type Conversion3/1 -> Communication/1
  Communication Loss/1 -> Logical Operator1/1
  Mux1/1 -> Mux/1
  Data Type Conversion5/1 -> Mux/4

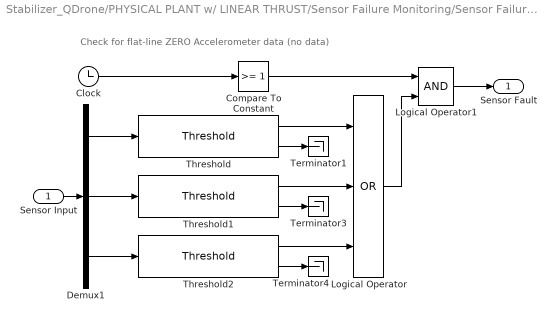
== system Stabilizer_QDrone/PHYSICAL PLANT w/ LINEAR THRUST/Sensor Failure Monitoring/Sensor Failure (Accelerometer) ==
  note: Check for flat-line ZERO Accelerometer data (no data)
  Sensor Input : Inport
  Clock : Clock
  Compare To Constant : simulink/Logic and Bit Operations/Compare To Constant  relop=>=  const=1  OutDataTypeStr=boolean
  Demux1 : Demux  Outputs=3
  Logical Operator : Logic  Operator=OR  Inputs=3  AllPortsSameDT=off  OutDataTypeStr=boolean
  Logical Operator1 : Logic  AllPortsSameDT=off  OutDataTypeStr=boolean
  Terminator1 : Terminator
  Terminator3 : Terminator
  Terminator4 : Terminator
  Threshold : quarc_library/Discontinuities/Threshold  operator===  param_src=Specify via dialog  threshold=0  duration=1
      settings: SourceProductName=The database C:\Users\user\AppData\Roaming\MathWorks\MATLAB\R2017a\slblocks_master.db is locked, or a table in the database is locked. (database is locked)
  Threshold1 : quarc_library/Discontinuities/Threshold  operator===  param_src=Specify via dialog  threshold=0  duration=1
      settings: SourceProductName=The database C:\Users\user\AppData\Roaming\MathWorks\MATLAB\R2017a\slblocks_master.db is locked, or a table in the database is locked. (database is locked)
  Threshold2 : quarc_library/Discontinuities/Threshold  operator===  param_src=Specify via dialog  threshold=0  duration=1
      settings: SourceProductName=The database C:\Users\user\AppData\Roaming\MathWorks\MATLAB\R2017a\slblocks_master.db is locked, or a table in the database is locked. (database is locked)
  Sensor Fault : Outport
  wires:
  Clock/1 -> Compare To Constant/1
  Threshold/1 -> Logical Operator/1
  Threshold1/1 -> Logical Operator/2
  Compare To Constant/1 -> Logical Operator1/1
  Logical Operator1/1 -> Sensor Fault/1
  Sensor Input/1 -> Demux1/1
  Threshold2/2 -> Terminator4/1
  Threshold2/1 -> Logical Operator/3
  Demux1/1 -> Threshold/1
  Demux1/3 -> Threshold2/1
  Demux1/2 -> Threshold1/1
  Logical Operator/1 -> Logical Operator1/2
  Threshold1/2 -> Terminator3/1
  Threshold/2 -> Terminator1/1

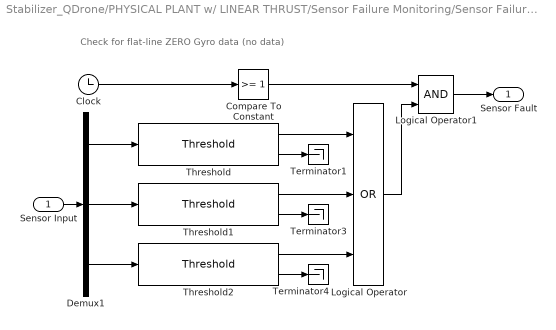
== system Stabilizer_QDrone/PHYSICAL PLANT w/ LINEAR THRUST/Sensor Failure Monitoring/Sensor Failure (Gyroscope) ==
  note: Check for flat-line ZERO Gyro data (no data)
  Sensor Input : Inport
  Clock : Clock
  Compare To Constant : simulink/Logic and Bit Operations/Compare To Constant  relop=>=  const=1  OutDataTypeStr=boolean
  Demux1 : Demux  Outputs=3
  Logical Operator : Logic  Operator=OR  Inputs=3  AllPortsSameDT=off  OutDataTypeStr=boolean
  Logical Operator1 : Logic  AllPortsSameDT=off  OutDataTypeStr=boolean
  Terminator1 : Terminator
  Terminator3 : Terminator
  Terminator4 : Terminator
  Threshold : quarc_library/Discontinuities/Threshold  operator===  param_src=Specify via dialog  threshold=0  duration=1
      settings: SourceProductName=The database C:\Users\user\AppData\Roaming\MathWorks\MATLAB\R2017a\slblocks_master.db is locked, or a table in the database is locked. (database is locked)
  Threshold1 : quarc_library/Discontinuities/Threshold  operator===  param_src=Specify via dialog  threshold=0  duration=1
      settings: SourceProductName=The database C:\Users\user\AppData\Roaming\MathWorks\MATLAB\R2017a\slblocks_master.db is locked, or a table in the database is locked. (database is locked)
  Threshold2 : quarc_library/Discontinuities/Threshold  operator===  param_src=Specify via dialog  threshold=0  duration=1
      settings: SourceProductName=The database C:\Users\user\AppData\Roaming\MathWorks\MATLAB\R2017a\slblocks_master.db is locked, or a table in the database is locked. (database is locked)
  Sensor Fault : Outport
  wires:
  Threshold/2 -> Terminator1/1
  Threshold1/2 -> Terminator3/1
  Logical Operator/1 -> Logical Operator1/2
  Demux1/2 -> Threshold1/1
  Demux1/3 -> Threshold2/1
  Demux1/1 -> Threshold/1
  Threshold2/1 -> Logical Operator/3
  Threshold2/2 -> Terminator4/1
  Sensor Input/1 -> Demux1/1
  Logical Operator1/1 -> Sensor Fault/1
  Compare To Constant/1 -> Logical Operator1/1
  Threshold1/1 -> Logical Operator/2
  Threshold/1 -> Logical Operator/1
  Clock/1 -> Compare To Constant/1

== matlab function PHYSICAL PLANT w// LINEAR THRUST/roll and pitch approximation from accelerometer ==
  data: roll_acc output double; pitch_acc output double; acc_body input double
function [roll_acc, pitch_acc]   = fcn(acc_body)
%#eml
n = norm(acc_body,2);
if n>eps
    acc_body = acc_body/n; 
else
    acc_body = [0 0 1]';
end

roll_acc = atan2(acc_body(2),acc_body(3));
pitch_acc = atan2( -acc_body(1), acc_body(2)*sin(roll_acc)+acc_body(3)*cos(roll_acc));

== matlab function Communication/Detect Communication loss/MATLAB Function ==
  settings: updateMethod=DISCRETE
  data: time input double; stream_connection_loss output double; state input double; error input double; ms_time input double; data_loss output double
function [stream_connection_loss , data_loss] = fcn(time, state, error, ms_time)
% signals(1) = throttle
% signals(2) = arm

persistent ms_time_prev
    if isempty(ms_time_prev)
        ms_time_prev = 0;
    end

stream_connection_loss = 0;
data_loss = 0;
if time > 3
    if ((state ~= 2)&&(error < 0))
        % stream connection is not established correctly
        stream_connection_loss = 1;
    end

    if (ms_time == ms_time_prev)
        % data is stale
        data_loss = 1;
    end
end

ms_time_prev = ms_time;

== matlab function PHYSICAL PLANT w// LINEAR THRUST/Red - Low Voltage Green - Armed Blue - Disarmed/MATLAB Function LED Color Assignment ==
  data: arm input double; value output double; low_battery input double
function value = fcn(arm, low_battery)

if low_battery
    value = 1;
elseif arm
    value = 2;
else 
    value = 3;
end
